simulink model "carpark_shuffler_sim"  (R2025b)
settings: Solver=VariableStepAuto  StartTime=0.0  StopTime=0.06  MaxStep=1e-4  RelTol=1e-4
PreLoadFcn:
  | init_params;
InitFcn:
  | init_params
undefined symbols (not defined in the file or in its folder): LOADP, SENSE, SRC
libraries: fl_lib x63, ee_lib x43, nesl_utility x37
(part 4 of 4)

== system carpark_shuffler_sim/Power Circuit/PV Module 1/power source/PV80 ==
  Diode : ee_lib/Semiconductors & Converters/Diode  ModelType=ee.enum.diode.modelType.pwl  TableType=ee.enum.diode.tableType.IfMat  IfMat=[.07, .12, .19, 1.75, 4.24, 7.32, 11.2; .16, .3, .72, 2.14, 5.02, 8.35, 13.12] A  VfMat=[.9, 1.15, 1.25, 1.5, 1.75, 2.17, 2.6, 2.85; .58, .68, .75, 1.1, 1.38, 1.77, 2.27, 2.7] V  TjVec=[25, 125] degC  VfVec=[.5, .7, .9, 1.3, 1.7, 2.1, 2.5] V  IfVec=[.1, .2, .5, 1, 2, 4, 7, 10] A  IrMat=[1e-06, 2e-06, 5e-06, 1e-05, 2.5e-05, 5e-05, .0001; 2e-06, 5e-06, 1e-05, 4e-05, 8e-05, .0002, .0005] A  VrMat=[10, 100, 200, 250, 300, 325, 350; 10, 70, 160, 220, 270, 300, 320] V  VrVec=[10, 20, 40, 50, 70, 80, 100] V  IrVec=[1e-06, 2e-06, 5e-06, 1e-05, 2e-05, 5e-05, .0001] A  Vf=0.6 V  Ron=0.3 Ohm  Goff=1e-8 S  prmExp=ee.enum.diode.expParam.useTwo  I12=[.0137, .545] A  V12=[.6, .7] V  RS=0 Ohm  Tmeas=298.15 K  IS=1e-12 A  ec=1  I1=0.0137 A  V1=0.6 V  N_series=1  N_parallel=1  ZenerEnable=false  Rz=0.3 Ohm  BV=inf V  C_param=ee.enum.diode.capParam.fixed  CJ=0 pF  CJ0=5 pF  Vvec=[.1, 10, 100] V  Cvec=[3.5, 1, .4] pF  VJ=1 V  Mgrad=0.5  FC=0.5  Q_param=ee.enum.diode.recoveryParam.off  iRM=-7.15 A  iF=4 A  didt=-750 A/us  trr_factor=3  trr=115 ns  Qrr=150 nA*s  Vr=-600 V  Ls=150 nH  Erec=0.03 J  TT=50 ns  tau=100 ns  T_param=ee.enum.diode.temperatureParam.off  Tdevice=298.15 K  I1_T2=0.245 A  V1_T2=0.5 V  IS_T2=1.25e-7 A  Tmeas2=125 degC  XTI_param=ee.enum.diode.xtiParam.pn  XTI=3  EG_param=ee.enum.diode.egapParam.material_si  EG=1.11 eV  dBVdT=0 V/K  enable_fault_input=simscape.enum.onoff.off  i_specify=off  i_priority=None  i=0 A  i_nominal_specify=off  i_nominal_value=1  i_nominal_unit=A  v_specify=off  v_priority=None  v=0 V  v_nominal_specify=off  v_nominal_value=1  v_nominal_unit=V  v_capacitor_specify=off  v_capacitor_priority=None  v_capacitor=0 V  v_capacitor_nominal_specify=off  v_capacitor_nominal_value=1  v_capacitor_nominal_unit=V  Qj_specify=off  Qj_priority=High  Qj=0 C  Qj_nominal_specify=off  Qj_nominal_value=1  Qj_nominal_unit=C  i_diode_specify=off  i_diode_priority=None  i_diode=0 A  i_diode_nominal_specify=off  i_diode_nominal_value=1  i_diode_nominal_unit=A  v_diode_specify=off  v_diode_priority=None  v_diode=0 V  v_diode_nominal_specify=off  v_diode_nominal_value=1  v_diode_nominal_unit=V  i_capacitor_specify=off  i_capacitor_priority=None  i_capacitor=0 A  i_capacitor_nominal_specify=off  i_capacitor_nominal_value=1  i_capacitor_nominal_unit=A  power_dissipated_specify=off  power_dissipated_priority=None  power_dissipated=0 W  power_dissipated_nominal_specify=off  power_dissipated_nominal_value=1  power_dissipated_nominal_unit=W  fidelity_level=ee.enum.diode.fidelity.includeChargeDyn  rec_loss_model=ee.enum.diode.reverseRecoveryModel.fixed  ErecVal=0 J  scaleWithIandV=true  ErecMat=zeros(2, 3) J  TjrecVec=[298.15, 398.15] K  IfrecVec=[.1, 1, 10] A  IrecVal=10 A  VrecVal=10 V  tFilter=1 / 1000 / 100 s  thermal_network_parameterization=ee.enum.thermalNetworkTopology.junctionCase  Rth=[0, 10] K/W  Rth_Cauer=[1, 3, 10] K/W  Rth_Foster=[.08, .14, .22, .16] K/W  thermal_mass_parameterization=ee.enum.thermalNetwork.timeconstant  thermal_mass=[0, 1] J/K  thermal_mass_Cauer=[.1, .3, 1] J/K  thermal_mass_Foster=[.001, .005, .05, .5] J/K  thermal_time_constant=[0, 10] s  thermal_time_constant_Cauer=[1, 3, 10] s  thermal_time_constant_Foster=[7e-05, .0007, .01, .08] s  thermal_mass_initial_temperatures=[25, 25] degC  thermal_mass_initial_temperatures_Cauer=[25, 25, 25] degC  junction_thermal_mass=0.01 J/K  Tvec_initial_Foster=[25, 25, 25, 25] degC  no_thermal_network=0  junction_temperature_specify=off  junction_temperature_priority=None  junction_temperature=25 degC  junction_temperature_nominal_specify=off  junction_temperature_nominal_value=1  junction_temperature_nominal_unit=degC
  Solar Cell : ee_lib/Sources/Solar Cell  prm=ee.enum.sources.solar_cell_prm.datasheet  Isc=SRC.pv80.Isc A  Voc=SRC.pv80.Voc_cell V  Is=1.728e-12 A  Is2=0 A  Iph=14.96 A  Ir0=1000 W/m^2  ec=1  N2=2  Rs=0.00263 Ohm  Rp=inf Ohm  N_series=SRC.pv80.Ns  N_parallel=1  TIPH1=0.0005 1/K  EG=1.11 eV  TXIS1=3  TXIS2=3  TRS1=0  TRP1=0  Tmeas=25 degC  TFIXED=25 degC  thermal_mass=100 J/K  initial_temperature=25 degC
  +ve : PMIOPort  Side=Left
  Irrad : PMIOPort  Port=2  Side=Left
  -ve : PMIOPort  Port=3  Side=Right
  connections:
  Solar Cell/LConn2 -- Diode/RConn1 -- +ve/RConn1
  -ve/RConn1 -- Solar Cell/RConn1 -- Diode/LConn1
  Irrad/RConn1 -- Solar Cell/LConn1

== system carpark_shuffler_sim/Power Circuit/PV Module 2/power source/BENCH ==
  Controlled Current Source : fl_lib/Electrical/Electrical Sources/Controlled Current Source
  DC Voltage Source : ee_lib/Additional Components/SPICE Sources/DC Voltage Source  DC=SRC.bench.Vset(1) V
  Diode : ee_lib/Semiconductors & Converters/Diode  ModelType=ee.enum.diode.modelType.pwl  TableType=ee.enum.diode.tableType.IfMat  IfMat=[.07, .12, .19, 1.75, 4.24, 7.32, 11.2; .16, .3, .72, 2.14, 5.02, 8.35, 13.12] A  VfMat=[.9, 1.15, 1.25, 1.5, 1.75, 2.17, 2.6, 2.85; .58, .68, .75, 1.1, 1.38, 1.77, 2.27, 2.7] V  TjVec=[25, 125] degC  VfVec=[.5, .7, .9, 1.3, 1.7, 2.1, 2.5] V  IfVec=[.1, .2, .5, 1, 2, 4, 7, 10] A  IrMat=[1e-06, 2e-06, 5e-06, 1e-05, 2.5e-05, 5e-05, .0001; 2e-06, 5e-06, 1e-05, 4e-05, 8e-05, .0002, .0005] A  VrMat=[10, 100, 200, 250, 300, 325, 350; 10, 70, 160, 220, 270, 300, 320] V  VrVec=[10, 20, 40, 50, 70, 80, 100] V  IrVec=[1e-06, 2e-06, 5e-06, 1e-05, 2e-05, 5e-05, .0001] A  Vf=1e-3 V  Ron=SRC.bench.Rclamp Ohm  Goff=1e-8 S  prmExp=ee.enum.diode.expParam.useTwo  I12=[.0137, .545] A  V12=[.6, .7] V  RS=0 Ohm  Tmeas=298.15 K  IS=1e-12 A  ec=1  I1=0.0137 A  V1=0.6 V  N_series=1  N_parallel=1  ZenerEnable=false  Rz=0.3 Ohm  BV=inf V  C_param=ee.enum.diode.capParam.fixed  CJ=0 pF  CJ0=5 pF  Vvec=[.1, 10, 100] V  Cvec=[3.5, 1, .4] pF  VJ=1 V  Mgrad=0.5  FC=0.5  Q_param=ee.enum.diode.recoveryParam.off  iRM=-7.15 A  iF=4 A  didt=-750 A/us  trr_factor=3  trr=115 ns  Qrr=150 nA*s  Vr=-600 V  Ls=150 nH  Erec=0.03 J  TT=50 ns  tau=100 ns  T_param=ee.enum.diode.temperatureParam.off  Tdevice=298.15 K  I1_T2=0.245 A  V1_T2=0.5 V  IS_T2=1.25e-7 A  Tmeas2=125 degC  XTI_param=ee.enum.diode.xtiParam.pn  XTI=3  EG_param=ee.enum.diode.egapParam.material_si  EG=1.11 eV  dBVdT=0 V/K  enable_fault_input=simscape.enum.onoff.off  i_specify=off  i_priority=None  i=0 A  i_nominal_specify=off  i_nominal_value=1  i_nominal_unit=A  v_specify=off  v_priority=None  v=0 V  v_nominal_specify=off  v_nominal_value=1  v_nominal_unit=V  v_capacitor_specify=off  v_capacitor_priority=None  v_capacitor=0 V  v_capacitor_nominal_specify=off  v_capacitor_nominal_value=1  v_capacitor_nominal_unit=V  Qj_specify=off  Qj_priority=High  Qj=0 C  Qj_nominal_specify=off  Qj_nominal_value=1  Qj_nominal_unit=C  i_diode_specify=off  i_diode_priority=None  i_diode=0 A  i_diode_nominal_specify=off  i_diode_nominal_value=1  i_diode_nominal_unit=A  v_diode_specify=off  v_diode_priority=None  v_diode=0 V  v_diode_nominal_specify=off  v_diode_nominal_value=1  v_diode_nominal_unit=V  i_capacitor_specify=off  i_capacitor_priority=None  i_capacitor=0 A  i_capacitor_nominal_specify=off  i_capacitor_nominal_value=1  i_capacitor_nominal_unit=A  power_dissipated_specify=off  power_dissipated_priority=None  power_dissipated=0 W  power_dissipated_nominal_specify=off  power_dissipated_nominal_value=1  power_dissipated_nominal_unit=W  fidelity_level=ee.enum.diode.fidelity.includeChargeDyn  rec_loss_model=ee.enum.diode.reverseRecoveryModel.fixed  ErecVal=0 J  scaleWithIandV=true  ErecMat=zeros(2, 3) J  TjrecVec=[298.15, 398.15] K  IfrecVec=[.1, 1, 10] A  IrecVal=10 A  VrecVal=10 V  tFilter=1 / 1000 / 100 s  thermal_network_parameterization=ee.enum.thermalNetworkTopology.junctionCase  Rth=[0, 10] K/W  Rth_Cauer=[1, 3, 10] K/W  Rth_Foster=[.08, .14, .22, .16] K/W  thermal_mass_parameterization=ee.enum.thermalNetwork.timeconstant  thermal_mass=[0, 1] J/K  thermal_mass_Cauer=[.1, .3, 1] J/K  thermal_mass_Foster=[.001, .005, .05, .5] J/K  thermal_time_constant=[0, 10] s  thermal_time_constant_Cauer=[1, 3, 10] s  thermal_time_constant_Foster=[7e-05, .0007, .01, .08] s  thermal_mass_initial_temperatures=[25, 25] degC  thermal_mass_initial_temperatures_Cauer=[25, 25, 25] degC  junction_thermal_mass=0.01 J/K  Tvec_initial_Foster=[25, 25, 25, 25] degC  no_thermal_network=0  junction_temperature_specify=off  junction_temperature_priority=None  junction_temperature=25 degC  junction_temperature_nominal_specify=off  junction_temperature_nominal_value=1  junction_temperature_nominal_unit=degC
  PS Gain : fl_lib/Physical Signals/Functions/PS Gain  gain=SRC.bench.Ilim(2)/1000
  Resistor : fl_lib/Electrical/Electrical Elements/Resistor  R=max(SRC.bench.Rs(1),1e-6) Ohm  i_specify=off  i_priority=None  i=0 A  i_nominal_specify=off  i_nominal_value=1  i_nominal_unit=A  v_specify=off  v_priority=None  v=0 V  v_nominal_specify=off  v_nominal_value=1  v_nominal_unit=V
  +ve : PMIOPort  Side=Left
  Irrad : PMIOPort  Port=2  Side=Left
  -ve : PMIOPort  Port=3  Side=Right
  connections:
  Resistor/RConn1 -- +ve/RConn1
  Controlled Current Source/RConn2 -- -ve/RConn1 -- DC Voltage Source/RConn1
  PS Gain/RConn1 -- Controlled Current Source/RConn1
  Controlled Current Source/LConn1 -- Resistor/LConn1 -- Diode/LConn1
  DC Voltage Source/LConn1 -- Diode/RConn1
  PS Gain/LConn1 -- Irrad/RConn1

== system carpark_shuffler_sim/Power Circuit/PV Module 2/power source/PV80 ==
  Diode : ee_lib/Semiconductors & Converters/Diode  ModelType=ee.enum.diode.modelType.pwl  TableType=ee.enum.diode.tableType.IfMat  IfMat=[.07, .12, .19, 1.75, 4.24, 7.32, 11.2; .16, .3, .72, 2.14, 5.02, 8.35, 13.12] A  VfMat=[.9, 1.15, 1.25, 1.5, 1.75, 2.17, 2.6, 2.85; .58, .68, .75, 1.1, 1.38, 1.77, 2.27, 2.7] V  TjVec=[25, 125] degC  VfVec=[.5, .7, .9, 1.3, 1.7, 2.1, 2.5] V  IfVec=[.1, .2, .5, 1, 2, 4, 7, 10] A  IrMat=[1e-06, 2e-06, 5e-06, 1e-05, 2.5e-05, 5e-05, .0001; 2e-06, 5e-06, 1e-05, 4e-05, 8e-05, .0002, .0005] A  VrMat=[10, 100, 200, 250, 300, 325, 350; 10, 70, 160, 220, 270, 300, 320] V  VrVec=[10, 20, 40, 50, 70, 80, 100] V  IrVec=[1e-06, 2e-06, 5e-06, 1e-05, 2e-05, 5e-05, .0001] A  Vf=0.6 V  Ron=0.3 Ohm  Goff=1e-8 S  prmExp=ee.enum.diode.expParam.useTwo  I12=[.0137, .545] A  V12=[.6, .7] V  RS=0 Ohm  Tmeas=298.15 K  IS=1e-12 A  ec=1  I1=0.0137 A  V1=0.6 V  N_series=1  N_parallel=1  ZenerEnable=false  Rz=0.3 Ohm  BV=inf V  C_param=ee.enum.diode.capParam.fixed  CJ=0 pF  CJ0=5 pF  Vvec=[.1, 10, 100] V  Cvec=[3.5, 1, .4] pF  VJ=1 V  Mgrad=0.5  FC=0.5  Q_param=ee.enum.diode.recoveryParam.off  iRM=-7.15 A  iF=4 A  didt=-750 A/us  trr_factor=3  trr=115 ns  Qrr=150 nA*s  Vr=-600 V  Ls=150 nH  Erec=0.03 J  TT=50 ns  tau=100 ns  T_param=ee.enum.diode.temperatureParam.off  Tdevice=298.15 K  I1_T2=0.245 A  V1_T2=0.5 V  IS_T2=1.25e-7 A  Tmeas2=125 degC  XTI_param=ee.enum.diode.xtiParam.pn  XTI=3  EG_param=ee.enum.diode.egapParam.material_si  EG=1.11 eV  dBVdT=0 V/K  enable_fault_input=simscape.enum.onoff.off  i_specify=off  i_priority=None  i=0 A  i_nominal_specify=off  i_nominal_value=1  i_nominal_unit=A  v_specify=off  v_priority=None  v=0 V  v_nominal_specify=off  v_nominal_value=1  v_nominal_unit=V  v_capacitor_specify=off  v_capacitor_priority=None  v_capacitor=0 V  v_capacitor_nominal_specify=off  v_capacitor_nominal_value=1  v_capacitor_nominal_unit=V  Qj_specify=off  Qj_priority=High  Qj=0 C  Qj_nominal_specify=off  Qj_nominal_value=1  Qj_nominal_unit=C  i_diode_specify=off  i_diode_priority=None  i_diode=0 A  i_diode_nominal_specify=off  i_diode_nominal_value=1  i_diode_nominal_unit=A  v_diode_specify=off  v_diode_priority=None  v_diode=0 V  v_diode_nominal_specify=off  v_diode_nominal_value=1  v_diode_nominal_unit=V  i_capacitor_specify=off  i_capacitor_priority=None  i_capacitor=0 A  i_capacitor_nominal_specify=off  i_capacitor_nominal_value=1  i_capacitor_nominal_unit=A  power_dissipated_specify=off  power_dissipated_priority=None  power_dissipated=0 W  power_dissipated_nominal_specify=off  power_dissipated_nominal_value=1  power_dissipated_nominal_unit=W  fidelity_level=ee.enum.diode.fidelity.includeChargeDyn  rec_loss_model=ee.enum.diode.reverseRecoveryModel.fixed  ErecVal=0 J  scaleWithIandV=true  ErecMat=zeros(2, 3) J  TjrecVec=[298.15, 398.15] K  IfrecVec=[.1, 1, 10] A  IrecVal=10 A  VrecVal=10 V  tFilter=1 / 1000 / 100 s  thermal_network_parameterization=ee.enum.thermalNetworkTopology.junctionCase  Rth=[0, 10] K/W  Rth_Cauer=[1, 3, 10] K/W  Rth_Foster=[.08, .14, .22, .16] K/W  thermal_mass_parameterization=ee.enum.thermalNetwork.timeconstant  thermal_mass=[0, 1] J/K  thermal_mass_Cauer=[.1, .3, 1] J/K  thermal_mass_Foster=[.001, .005, .05, .5] J/K  thermal_time_constant=[0, 10] s  thermal_time_constant_Cauer=[1, 3, 10] s  thermal_time_constant_Foster=[7e-05, .0007, .01, .08] s  thermal_mass_initial_temperatures=[25, 25] degC  thermal_mass_initial_temperatures_Cauer=[25, 25, 25] degC  junction_thermal_mass=0.01 J/K  Tvec_initial_Foster=[25, 25, 25, 25] degC  no_thermal_network=0  junction_temperature_specify=off  junction_temperature_priority=None  junction_temperature=25 degC  junction_temperature_nominal_specify=off  junction_temperature_nominal_value=1  junction_temperature_nominal_unit=degC
  Solar Cell : ee_lib/Sources/Solar Cell  prm=ee.enum.sources.solar_cell_prm.datasheet  Isc=SRC.pv80.Isc A  Voc=SRC.pv80.Voc_cell V  Is=1.728e-12 A  Is2=0 A  Iph=14.96 A  Ir0=1000 W/m^2  ec=1  N2=2  Rs=0.00263 Ohm  Rp=inf Ohm  N_series=SRC.pv80.Ns  N_parallel=1  TIPH1=0.0005 1/K  EG=1.11 eV  TXIS1=3  TXIS2=3  TRS1=0  TRP1=0  Tmeas=25 degC  TFIXED=25 degC  thermal_mass=100 J/K  initial_temperature=25 degC
  +ve : PMIOPort  Side=Left
  Irrad : PMIOPort  Port=2  Side=Left
  -ve : PMIOPort  Port=3  Side=Right
  connections:
  Diode/RConn1 -- Solar Cell/LConn2 -- +ve/RConn1
  Diode/LConn1 -- -ve/RConn1 -- Solar Cell/RConn1
  Irrad/RConn1 -- Solar Cell/LConn1

== system carpark_shuffler_sim/Power Circuit/PV Module 3/power source/BENCH ==
  Controlled Current Source : fl_lib/Electrical/Electrical Sources/Controlled Current Source
  DC Voltage Source : ee_lib/Additional Components/SPICE Sources/DC Voltage Source  DC=SRC.bench.Vset(1) V
  Diode : ee_lib/Semiconductors & Converters/Diode  ModelType=ee.enum.diode.modelType.pwl  TableType=ee.enum.diode.tableType.IfMat  IfMat=[.07, .12, .19, 1.75, 4.24, 7.32, 11.2; .16, .3, .72, 2.14, 5.02, 8.35, 13.12] A  VfMat=[.9, 1.15, 1.25, 1.5, 1.75, 2.17, 2.6, 2.85; .58, .68, .75, 1.1, 1.38, 1.77, 2.27, 2.7] V  TjVec=[25, 125] degC  VfVec=[.5, .7, .9, 1.3, 1.7, 2.1, 2.5] V  IfVec=[.1, .2, .5, 1, 2, 4, 7, 10] A  IrMat=[1e-06, 2e-06, 5e-06, 1e-05, 2.5e-05, 5e-05, .0001; 2e-06, 5e-06, 1e-05, 4e-05, 8e-05, .0002, .0005] A  VrMat=[10, 100, 200, 250, 300, 325, 350; 10, 70, 160, 220, 270, 300, 320] V  VrVec=[10, 20, 40, 50, 70, 80, 100] V  IrVec=[1e-06, 2e-06, 5e-06, 1e-05, 2e-05, 5e-05, .0001] A  Vf=1e-3 V  Ron=SRC.bench.Rclamp Ohm  Goff=1e-8 S  prmExp=ee.enum.diode.expParam.useTwo  I12=[.0137, .545] A  V12=[.6, .7] V  RS=0 Ohm  Tmeas=298.15 K  IS=1e-12 A  ec=1  I1=0.0137 A  V1=0.6 V  N_series=1  N_parallel=1  ZenerEnable=false  Rz=0.3 Ohm  BV=inf V  C_param=ee.enum.diode.capParam.fixed  CJ=0 pF  CJ0=5 pF  Vvec=[.1, 10, 100] V  Cvec=[3.5, 1, .4] pF  VJ=1 V  Mgrad=0.5  FC=0.5  Q_param=ee.enum.diode.recoveryParam.off  iRM=-7.15 A  iF=4 A  didt=-750 A/us  trr_factor=3  trr=115 ns  Qrr=150 nA*s  Vr=-600 V  Ls=150 nH  Erec=0.03 J  TT=50 ns  tau=100 ns  T_param=ee.enum.diode.temperatureParam.off  Tdevice=298.15 K  I1_T2=0.245 A  V1_T2=0.5 V  IS_T2=1.25e-7 A  Tmeas2=125 degC  XTI_param=ee.enum.diode.xtiParam.pn  XTI=3  EG_param=ee.enum.diode.egapParam.material_si  EG=1.11 eV  dBVdT=0 V/K  enable_fault_input=simscape.enum.onoff.off  i_specify=off  i_priority=None  i=0 A  i_nominal_specify=off  i_nominal_value=1  i_nominal_unit=A  v_specify=off  v_priority=None  v=0 V  v_nominal_specify=off  v_nominal_value=1  v_nominal_unit=V  v_capacitor_specify=off  v_capacitor_priority=None  v_capacitor=0 V  v_capacitor_nominal_specify=off  v_capacitor_nominal_value=1  v_capacitor_nominal_unit=V  Qj_specify=off  Qj_priority=High  Qj=0 C  Qj_nominal_specify=off  Qj_nominal_value=1  Qj_nominal_unit=C  i_diode_specify=off  i_diode_priority=None  i_diode=0 A  i_diode_nominal_specify=off  i_diode_nominal_value=1  i_diode_nominal_unit=A  v_diode_specify=off  v_diode_priority=None  v_diode=0 V  v_diode_nominal_specify=off  v_diode_nominal_value=1  v_diode_nominal_unit=V  i_capacitor_specify=off  i_capacitor_priority=None  i_capacitor=0 A  i_capacitor_nominal_specify=off  i_capacitor_nominal_value=1  i_capacitor_nominal_unit=A  power_dissipated_specify=off  power_dissipated_priority=None  power_dissipated=0 W  power_dissipated_nominal_specify=off  power_dissipated_nominal_value=1  power_dissipated_nominal_unit=W  fidelity_level=ee.enum.diode.fidelity.includeChargeDyn  rec_loss_model=ee.enum.diode.reverseRecoveryModel.fixed  ErecVal=0 J  scaleWithIandV=true  ErecMat=zeros(2, 3) J  TjrecVec=[298.15, 398.15] K  IfrecVec=[.1, 1, 10] A  IrecVal=10 A  VrecVal=10 V  tFilter=1 / 1000 / 100 s  thermal_network_parameterization=ee.enum.thermalNetworkTopology.junctionCase  Rth=[0, 10] K/W  Rth_Cauer=[1, 3, 10] K/W  Rth_Foster=[.08, .14, .22, .16] K/W  thermal_mass_parameterization=ee.enum.thermalNetwork.timeconstant  thermal_mass=[0, 1] J/K  thermal_mass_Cauer=[.1, .3, 1] J/K  thermal_mass_Foster=[.001, .005, .05, .5] J/K  thermal_time_constant=[0, 10] s  thermal_time_constant_Cauer=[1, 3, 10] s  thermal_time_constant_Foster=[7e-05, .0007, .01, .08] s  thermal_mass_initial_temperatures=[25, 25] degC  thermal_mass_initial_temperatures_Cauer=[25, 25, 25] degC  junction_thermal_mass=0.01 J/K  Tvec_initial_Foster=[25, 25, 25, 25] degC  no_thermal_network=0  junction_temperature_specify=off  junction_temperature_priority=None  junction_temperature=25 degC  junction_temperature_nominal_specify=off  junction_temperature_nominal_value=1  junction_temperature_nominal_unit=degC
  PS Gain : fl_lib/Physical Signals/Functions/PS Gain  gain=SRC.bench.Ilim(3)/1000
  Resistor : fl_lib/Electrical/Electrical Elements/Resistor  R=max(SRC.bench.Rs(1),1e-6) Ohm  i_specify=off  i_priority=None  i=0 A  i_nominal_specify=off  i_nominal_value=1  i_nominal_unit=A  v_specify=off  v_priority=None  v=0 V  v_nominal_specify=off  v_nominal_value=1  v_nominal_unit=V
  +ve : PMIOPort  Side=Left
  Irrad : PMIOPort  Port=2  Side=Left
  -ve : PMIOPort  Port=3  Side=Right
  connections:
  Resistor/RConn1 -- +ve/RConn1
  Controlled Current Source/RConn2 -- -ve/RConn1 -- DC Voltage Source/RConn1
  PS Gain/RConn1 -- Controlled Current Source/RConn1
  Controlled Current Source/LConn1 -- Resistor/LConn1 -- Diode/LConn1
  DC Voltage Source/LConn1 -- Diode/RConn1
  PS Gain/LConn1 -- Irrad/RConn1

== system carpark_shuffler_sim/Power Circuit/PV Module 3/power source/PV80 ==
  Diode : ee_lib/Semiconductors & Converters/Diode  ModelType=ee.enum.diode.modelType.pwl  TableType=ee.enum.diode.tableType.IfMat  IfMat=[.07, .12, .19, 1.75, 4.24, 7.32, 11.2; .16, .3, .72, 2.14, 5.02, 8.35, 13.12] A  VfMat=[.9, 1.15, 1.25, 1.5, 1.75, 2.17, 2.6, 2.85; .58, .68, .75, 1.1, 1.38, 1.77, 2.27, 2.7] V  TjVec=[25, 125] degC  VfVec=[.5, .7, .9, 1.3, 1.7, 2.1, 2.5] V  IfVec=[.1, .2, .5, 1, 2, 4, 7, 10] A  IrMat=[1e-06, 2e-06, 5e-06, 1e-05, 2.5e-05, 5e-05, .0001; 2e-06, 5e-06, 1e-05, 4e-05, 8e-05, .0002, .0005] A  VrMat=[10, 100, 200, 250, 300, 325, 350; 10, 70, 160, 220, 270, 300, 320] V  VrVec=[10, 20, 40, 50, 70, 80, 100] V  IrVec=[1e-06, 2e-06, 5e-06, 1e-05, 2e-05, 5e-05, .0001] A  Vf=0.6 V  Ron=0.3 Ohm  Goff=1e-8 S  prmExp=ee.enum.diode.expParam.useTwo  I12=[.0137, .545] A  V12=[.6, .7] V  RS=0 Ohm  Tmeas=298.15 K  IS=1e-12 A  ec=1  I1=0.0137 A  V1=0.6 V  N_series=1  N_parallel=1  ZenerEnable=false  Rz=0.3 Ohm  BV=inf V  C_param=ee.enum.diode.capParam.fixed  CJ=0 pF  CJ0=5 pF  Vvec=[.1, 10, 100] V  Cvec=[3.5, 1, .4] pF  VJ=1 V  Mgrad=0.5  FC=0.5  Q_param=ee.enum.diode.recoveryParam.off  iRM=-7.15 A  iF=4 A  didt=-750 A/us  trr_factor=3  trr=115 ns  Qrr=150 nA*s  Vr=-600 V  Ls=150 nH  Erec=0.03 J  TT=50 ns  tau=100 ns  T_param=ee.enum.diode.temperatureParam.off  Tdevice=298.15 K  I1_T2=0.245 A  V1_T2=0.5 V  IS_T2=1.25e-7 A  Tmeas2=125 degC  XTI_param=ee.enum.diode.xtiParam.pn  XTI=3  EG_param=ee.enum.diode.egapParam.material_si  EG=1.11 eV  dBVdT=0 V/K  enable_fault_input=simscape.enum.onoff.off  i_specify=off  i_priority=None  i=0 A  i_nominal_specify=off  i_nominal_value=1  i_nominal_unit=A  v_specify=off  v_priority=None  v=0 V  v_nominal_specify=off  v_nominal_value=1  v_nominal_unit=V  v_capacitor_specify=off  v_capacitor_priority=None  v_capacitor=0 V  v_capacitor_nominal_specify=off  v_capacitor_nominal_value=1  v_capacitor_nominal_unit=V  Qj_specify=off  Qj_priority=High  Qj=0 C  Qj_nominal_specify=off  Qj_nominal_value=1  Qj_nominal_unit=C  i_diode_specify=off  i_diode_priority=None  i_diode=0 A  i_diode_nominal_specify=off  i_diode_nominal_value=1  i_diode_nominal_unit=A  v_diode_specify=off  v_diode_priority=None  v_diode=0 V  v_diode_nominal_specify=off  v_diode_nominal_value=1  v_diode_nominal_unit=V  i_capacitor_specify=off  i_capacitor_priority=None  i_capacitor=0 A  i_capacitor_nominal_specify=off  i_capacitor_nominal_value=1  i_capacitor_nominal_unit=A  power_dissipated_specify=off  power_dissipated_priority=None  power_dissipated=0 W  power_dissipated_nominal_specify=off  power_dissipated_nominal_value=1  power_dissipated_nominal_unit=W  fidelity_level=ee.enum.diode.fidelity.includeChargeDyn  rec_loss_model=ee.enum.diode.reverseRecoveryModel.fixed  ErecVal=0 J  scaleWithIandV=true  ErecMat=zeros(2, 3) J  TjrecVec=[298.15, 398.15] K  IfrecVec=[.1, 1, 10] A  IrecVal=10 A  VrecVal=10 V  tFilter=1 / 1000 / 100 s  thermal_network_parameterization=ee.enum.thermalNetworkTopology.junctionCase  Rth=[0, 10] K/W  Rth_Cauer=[1, 3, 10] K/W  Rth_Foster=[.08, .14, .22, .16] K/W  thermal_mass_parameterization=ee.enum.thermalNetwork.timeconstant  thermal_mass=[0, 1] J/K  thermal_mass_Cauer=[.1, .3, 1] J/K  thermal_mass_Foster=[.001, .005, .05, .5] J/K  thermal_time_constant=[0, 10] s  thermal_time_constant_Cauer=[1, 3, 10] s  thermal_time_constant_Foster=[7e-05, .0007, .01, .08] s  thermal_mass_initial_temperatures=[25, 25] degC  thermal_mass_initial_temperatures_Cauer=[25, 25, 25] degC  junction_thermal_mass=0.01 J/K  Tvec_initial_Foster=[25, 25, 25, 25] degC  no_thermal_network=0  junction_temperature_specify=off  junction_temperature_priority=None  junction_temperature=25 degC  junction_temperature_nominal_specify=off  junction_temperature_nominal_value=1  junction_temperature_nominal_unit=degC
  Solar Cell : ee_lib/Sources/Solar Cell  prm=ee.enum.sources.solar_cell_prm.datasheet  Isc=SRC.pv80.Isc A  Voc=SRC.pv80.Voc_cell V  Is=1.728e-12 A  Is2=0 A  Iph=14.96 A  Ir0=1000 W/m^2  ec=1  N2=2  Rs=0.00263 Ohm  Rp=inf Ohm  N_series=SRC.pv80.Ns  N_parallel=1  TIPH1=0.0005 1/K  EG=1.11 eV  TXIS1=3  TXIS2=3  TRS1=0  TRP1=0  Tmeas=25 degC  TFIXED=25 degC  thermal_mass=100 J/K  initial_temperature=25 degC
  +ve : PMIOPort  Side=Left
  Irrad : PMIOPort  Port=2  Side=Left
  -ve : PMIOPort  Port=3  Side=Right
  connections:
  Diode/RConn1 -- Solar Cell/LConn2 -- +ve/RConn1
  Diode/LConn1 -- -ve/RConn1 -- Solar Cell/RConn1
  Irrad/RConn1 -- Solar Cell/LConn1

== system carpark_shuffler_sim/Power Circuit/Power Shuffler1/Phase A Half Bridge/Phase A Gate Driver ==
  A Control : Inport
  Controlled PWM Voltage : ee_lib/Integrated Circuits/Controlled PWM Voltage  F=200 kHz  TD=0 s  pulse_width_offset=0 s  pulse_min=0 s  pwm_or_av=ee.enum.pwm_or_av.pwm  event_type=ee.enum.ic.event.asynchronous  sample_time=1e-6 s  Vmin=0 V  Vmax=5 V  Vm=5 V  u_min=0  u_max=1
      settings: InternalSimscapePortConfiguration="{\"Bottom\":[],\"Left\":[{\"id\":\"u\",\"label\":\"u\",\"type\":\"input\"}],\"Right\":[{\"id\":\"p2\",\"label\":\"PWM\",\"type\":\"foundation.electrical.electrical\"},{\"id\":\"n2\",\"label\":\"REF\",\"type\":\"foundation.electrical.electrical\"}],\"Top\":[]}"
  Electrical Reference : fl_lib/Electrical/Electrical Elements/Electrical Reference
  Electrical Reference1 : fl_lib/Electrical/Electrical Elements/Electrical Reference
  Half-Bridge Driver : ee_lib/Semiconductors & Converters/Half-Bridge Driver  port_option=ee.enum.controlport.elec  uHigh=2.0 V  uLow=0.8 V  uHighValue=0.7  uLowValue=0.3  vHigh=15 V  vLow=0 V  tpLH=50 ns  tdLH=100 ns  tpHL=50 ns  tdHL=100 ns  parameterization=ee.enum.semiconductors.gateDriverParam.outputImpedance  rHigh=2 Ohm  rLow=2 Ohm  tRise=20 ns  tFall=20 ns  cLoad=10 nF  ZonTime_specify=off  ZonTime_priority=None  ZonTime=0 s  ZoffTime_specify=off  ZoffTime_priority=None  ZoffTime=0 s  power_dissipated_high_side_specify=off  power_dissipated_high_side_priority=None  power_dissipated_high_side=0 W  power_dissipated_high_side_nominal_specify=off  power_dissipated_high_side_nominal_value=1  power_dissipated_high_side_nominal_unit=W  power_dissipated_low_side_specify=off  power_dissipated_low_side_priority=None  power_dissipated_low_side=0 W  power_dissipated_low_side_nominal_specify=off  power_dissipated_low_side_nominal_value=1  power_dissipated_low_side_nominal_unit=W
      settings: InternalSimscapePortConfiguration="{\"Bottom\":[],\"Left\":[{\"id\":\"PWM\",\"label\":\"PWM\",\"type\":\"foundation.electrical.electrical\"},{\"id\":\"REF\",\"label\":\"REF\",\"type\":\"foundation.electrical.electrical\"}],\"Right\":[{\"id\":\"HO\",\"label\":\"HO\",\"type\":\"foundation.electrical.electrical\"},{\"id\":\"HS\",\"label\":\"HS\",\"type\":\"foundation.electrical.electrical\"},{\"id\":\"LO\",\"label\":\"LO\",\"type\":\"foundation.electrical.electrical\"},{\"id\":\"LS\",\"label\":\"LS\",\"type\":\"foundation.electrical.electrical\"}],\"Top\":[]}"
  Simulink-PS Converter1 : nesl_utility/Simulink-PS Converter  PhysicalDomain=network_engine_domain  SubClassName=ps_input  LeftPortType=input  RightPortType=output  PseudoPeriodic=off  Frequencies=[]  NoiseDistribution=none  NoiseParameters=[]  Unit=1  AffineConversion=off  FilteringAndDerivatives=provide  SimscapeFilterOrder=1  InputFilterTimeConstant=0.001  UdotUserProvided=0
  PWMH : PMIOPort  Side=Right
  phase : PMIOPort  Port=2  Side=Right
  PWML : PMIOPort  Port=3  Side=Right
  wires:
  A Control/1 -> Simulink-PS Converter1/1
  connections:
  Half-Bridge Driver/LConn2 -- Electrical Reference1/LConn1 -- Controlled PWM Voltage/RConn2
  Simulink-PS Converter1/RConn1 -- Controlled PWM Voltage/LConn1
  Half-Bridge Driver/RConn3 -- PWML/RConn1
  Electrical Reference/LConn1 -- Half-Bridge Driver/RConn4
  Half-Bridge Driver/RConn2 -- phase/RConn1
  Half-Bridge Driver/RConn1 -- PWMH/RConn1
  Controlled PWM Voltage/RConn1 -- Half-Bridge Driver/LConn1

== system carpark_shuffler_sim/Power Circuit/Power Shuffler1/Phase B Half Bridge/Phase B Gate Driver ==
  B Control : Inport
  Controlled PWM Voltage : ee_lib/Integrated Circuits/Controlled PWM Voltage  F=200 kHz  TD=1/(2 *200000) s  pulse_width_offset=0 s  pulse_min=0 s  pwm_or_av=ee.enum.pwm_or_av.pwm  event_type=ee.enum.ic.event.asynchronous  sample_time=1e-6 s  Vmin=0 V  Vmax=5 V  Vm=5 V  u_min=0  u_max=1
      settings: InternalSimscapePortConfiguration="{\"Bottom\":[],\"Left\":[{\"id\":\"u\",\"label\":\"u\",\"type\":\"input\"}],\"Right\":[{\"id\":\"p2\",\"label\":\"PWM\",\"type\":\"foundation.electrical.electrical\"},{\"id\":\"n2\",\"label\":\"REF\",\"type\":\"foundation.electrical.electrical\"}],\"Top\":[]}"
  Electrical Reference : fl_lib/Electrical/Electrical Elements/Electrical Reference
  Electrical Reference1 : fl_lib/Electrical/Electrical Elements/Electrical Reference
  Half-Bridge Driver : ee_lib/Semiconductors & Converters/Half-Bridge Driver  port_option=ee.enum.controlport.elec  uHigh=2.0 V  uLow=0.8 V  uHighValue=0.7  uLowValue=0.3  vHigh=15 V  vLow=0 V  tpLH=50 ns  tdLH=100 ns  tpHL=50 ns  tdHL=100 ns  parameterization=ee.enum.semiconductors.gateDriverParam.outputImpedance  rHigh=2 Ohm  rLow=2 Ohm  tRise=20 ns  tFall=20 ns  cLoad=10 nF  ZonTime_specify=off  ZonTime_priority=None  ZonTime=0 s  ZoffTime_specify=off  ZoffTime_priority=None  ZoffTime=0 s  power_dissipated_high_side_specify=off  power_dissipated_high_side_priority=None  power_dissipated_high_side=0 W  power_dissipated_high_side_nominal_specify=off  power_dissipated_high_side_nominal_value=1  power_dissipated_high_side_nominal_unit=W  power_dissipated_low_side_specify=off  power_dissipated_low_side_priority=None  power_dissipated_low_side=0 W  power_dissipated_low_side_nominal_specify=off  power_dissipated_low_side_nominal_value=1  power_dissipated_low_side_nominal_unit=W
      settings: InternalSimscapePortConfiguration="{\"Bottom\":[],\"Left\":[{\"id\":\"PWM\",\"label\":\"PWM\",\"type\":\"foundation.electrical.electrical\"},{\"id\":\"REF\",\"label\":\"REF\",\"type\":\"foundation.electrical.electrical\"}],\"Right\":[{\"id\":\"HO\",\"label\":\"HO\",\"type\":\"foundation.electrical.electrical\"},{\"id\":\"HS\",\"label\":\"HS\",\"type\":\"foundation.electrical.electrical\"},{\"id\":\"LO\",\"label\":\"LO\",\"type\":\"foundation.electrical.electrical\"},{\"id\":\"LS\",\"label\":\"LS\",\"type\":\"foundation.electrical.electrical\"}],\"Top\":[]}"
  Simulink-PS Converter1 : nesl_utility/Simulink-PS Converter  PhysicalDomain=network_engine_domain  SubClassName=ps_input  LeftPortType=input  RightPortType=output  PseudoPeriodic=off  Frequencies=[]  NoiseDistribution=none  NoiseParameters=[]  Unit=1  AffineConversion=off  FilteringAndDerivatives=provide  SimscapeFilterOrder=1  InputFilterTimeConstant=0.001  UdotUserProvided=0
  PWMH : PMIOPort  Side=Right
  phase : PMIOPort  Port=2  Side=Right
  PWML : PMIOPort  Port=3  Side=Right
  wires:
  B Control/1 -> Simulink-PS Converter1/1
  connections:
  Half-Bridge Driver/RConn2 -- phase/RConn1
  Half-Bridge Driver/RConn1 -- PWMH/RConn1
  Half-Bridge Driver/RConn3 -- PWML/RConn1
  Electrical Reference/LConn1 -- Half-Bridge Driver/RConn4
  Simulink-PS Converter1/RConn1 -- Controlled PWM Voltage/LConn1
  Controlled PWM Voltage/RConn1 -- Half-Bridge Driver/LConn1
  Electrical Reference1/LConn1 -- Controlled PWM Voltage/RConn2 -- Half-Bridge Driver/LConn2

== system carpark_shuffler_sim/Power Circuit/Power Shuffler2/Phase A Half Bridge/Phase A Gate Driver ==
  A Control : Inport
  Controlled PWM Voltage : ee_lib/Integrated Circuits/Controlled PWM Voltage  F=200 kHz  TD=0 s  pulse_width_offset=0 s  pulse_min=0 s  pwm_or_av=ee.enum.pwm_or_av.pwm  event_type=ee.enum.ic.event.asynchronous  sample_time=1e-6 s  Vmin=0 V  Vmax=5 V  Vm=5 V  u_min=0  u_max=1
      settings: InternalSimscapePortConfiguration="{\"Bottom\":[],\"Left\":[{\"id\":\"u\",\"label\":\"u\",\"type\":\"input\"}],\"Right\":[{\"id\":\"p2\",\"label\":\"PWM\",\"type\":\"foundation.electrical.electrical\"},{\"id\":\"n2\",\"label\":\"REF\",\"type\":\"foundation.electrical.electrical\"}],\"Top\":[]}"
  Electrical Reference : fl_lib/Electrical/Electrical Elements/Electrical Reference
  Electrical Reference1 : fl_lib/Electrical/Electrical Elements/Electrical Reference
  Half-Bridge Driver : ee_lib/Semiconductors & Converters/Half-Bridge Driver  port_option=ee.enum.controlport.elec  uHigh=2.0 V  uLow=0.8 V  uHighValue=0.7  uLowValue=0.3  vHigh=15 V  vLow=0 V  tpLH=50 ns  tdLH=100 ns  tpHL=50 ns  tdHL=100 ns  parameterization=ee.enum.semiconductors.gateDriverParam.outputImpedance  rHigh=2 Ohm  rLow=2 Ohm  tRise=20 ns  tFall=20 ns  cLoad=10 nF  ZonTime_specify=off  ZonTime_priority=None  ZonTime=0 s  ZoffTime_specify=off  ZoffTime_priority=None  ZoffTime=0 s  power_dissipated_high_side_specify=off  power_dissipated_high_side_priority=None  power_dissipated_high_side=0 W  power_dissipated_high_side_nominal_specify=off  power_dissipated_high_side_nominal_value=1  power_dissipated_high_side_nominal_unit=W  power_dissipated_low_side_specify=off  power_dissipated_low_side_priority=None  power_dissipated_low_side=0 W  power_dissipated_low_side_nominal_specify=off  power_dissipated_low_side_nominal_value=1  power_dissipated_low_side_nominal_unit=W
      settings: InternalSimscapePortConfiguration="{\"Bottom\":[],\"Left\":[{\"id\":\"PWM\",\"label\":\"PWM\",\"type\":\"foundation.electrical.electrical\"},{\"id\":\"REF\",\"label\":\"REF\",\"type\":\"foundation.electrical.electrical\"}],\"Right\":[{\"id\":\"HO\",\"label\":\"HO\",\"type\":\"foundation.electrical.electrical\"},{\"id\":\"HS\",\"label\":\"HS\",\"type\":\"foundation.electrical.electrical\"},{\"id\":\"LO\",\"label\":\"LO\",\"type\":\"foundation.electrical.electrical\"},{\"id\":\"LS\",\"label\":\"LS\",\"type\":\"foundation.electrical.electrical\"}],\"Top\":[]}"
  Simulink-PS Converter1 : nesl_utility/Simulink-PS Converter  PhysicalDomain=network_engine_domain  SubClassName=ps_input  LeftPortType=input  RightPortType=output  PseudoPeriodic=off  Frequencies=[]  NoiseDistribution=none  NoiseParameters=[]  Unit=1  AffineConversion=off  FilteringAndDerivatives=provide  SimscapeFilterOrder=1  InputFilterTimeConstant=0.001  UdotUserProvided=0
  PWMH : PMIOPort  Side=Right
  phase : PMIOPort  Port=2  Side=Right
  PWML : PMIOPort  Port=3  Side=Right
  wires:
  A Control/1 -> Simulink-PS Converter1/1
  connections:
  Half-Bridge Driver/LConn2 -- Electrical Reference1/LConn1 -- Controlled PWM Voltage/RConn2
  Simulink-PS Converter1/RConn1 -- Controlled PWM Voltage/LConn1
  Half-Bridge Driver/RConn3 -- PWML/RConn1
  Electrical Reference/LConn1 -- Half-Bridge Driver/RConn4
  Half-Bridge Driver/RConn2 -- phase/RConn1
  Half-Bridge Driver/RConn1 -- PWMH/RConn1
  Controlled PWM Voltage/RConn1 -- Half-Bridge Driver/LConn1

== system carpark_shuffler_sim/Power Circuit/Power Shuffler2/Phase B Half Bridge/Phase B Gate Driver ==
  B Control : Inport
  Controlled PWM Voltage : ee_lib/Integrated Circuits/Controlled PWM Voltage  F=200 kHz  TD=1/(2 *200000) s  pulse_width_offset=0 s  pulse_min=0 s  pwm_or_av=ee.enum.pwm_or_av.pwm  event_type=ee.enum.ic.event.asynchronous  sample_time=1e-6 s  Vmin=0 V  Vmax=5 V  Vm=5 V  u_min=0  u_max=1
      settings: InternalSimscapePortConfiguration="{\"Bottom\":[],\"Left\":[{\"id\":\"u\",\"label\":\"u\",\"type\":\"input\"}],\"Right\":[{\"id\":\"p2\",\"label\":\"PWM\",\"type\":\"foundation.electrical.electrical\"},{\"id\":\"n2\",\"label\":\"REF\",\"type\":\"foundation.electrical.electrical\"}],\"Top\":[]}"
  Electrical Reference : fl_lib/Electrical/Electrical Elements/Electrical Reference
  Electrical Reference1 : fl_lib/Electrical/Electrical Elements/Electrical Reference
  Half-Bridge Driver : ee_lib/Semiconductors & Converters/Half-Bridge Driver  port_option=ee.enum.controlport.elec  uHigh=2.0 V  uLow=0.8 V  uHighValue=0.7  uLowValue=0.3  vHigh=15 V  vLow=0 V  tpLH=50 ns  tdLH=100 ns  tpHL=50 ns  tdHL=100 ns  parameterization=ee.enum.semiconductors.gateDriverParam.outputImpedance  rHigh=2 Ohm  rLow=2 Ohm  tRise=20 ns  tFall=20 ns  cLoad=10 nF  ZonTime_specify=off  ZonTime_priority=None  ZonTime=0 s  ZoffTime_specify=off  ZoffTime_priority=None  ZoffTime=0 s  power_dissipated_high_side_specify=off  power_dissipated_high_side_priority=None  power_dissipated_high_side=0 W  power_dissipated_high_side_nominal_specify=off  power_dissipated_high_side_nominal_value=1  power_dissipated_high_side_nominal_unit=W  power_dissipated_low_side_specify=off  power_dissipated_low_side_priority=None  power_dissipated_low_side=0 W  power_dissipated_low_side_nominal_specify=off  power_dissipated_low_side_nominal_value=1  power_dissipated_low_side_nominal_unit=W
      settings: InternalSimscapePortConfiguration="{\"Bottom\":[],\"Left\":[{\"id\":\"PWM\",\"label\":\"PWM\",\"type\":\"foundation.electrical.electrical\"},{\"id\":\"REF\",\"label\":\"REF\",\"type\":\"foundation.electrical.electrical\"}],\"Right\":[{\"id\":\"HO\",\"label\":\"HO\",\"type\":\"foundation.electrical.electrical\"},{\"id\":\"HS\",\"label\":\"HS\",\"type\":\"foundation.electrical.electrical\"},{\"id\":\"LO\",\"label\":\"LO\",\"type\":\"foundation.electrical.electrical\"},{\"id\":\"LS\",\"label\":\"LS\",\"type\":\"foundation.electrical.electrical\"}],\"Top\":[]}"
  Simulink-PS Converter1 : nesl_utility/Simulink-PS Converter  PhysicalDomain=network_engine_domain  SubClassName=ps_input  LeftPortType=input  RightPortType=output  PseudoPeriodic=off  Frequencies=[]  NoiseDistribution=none  NoiseParameters=[]  Unit=1  AffineConversion=off  FilteringAndDerivatives=provide  SimscapeFilterOrder=1  InputFilterTimeConstant=0.001  UdotUserProvided=0
  PWMH : PMIOPort  Side=Right
  phase : PMIOPort  Port=2  Side=Right
  PWML : PMIOPort  Port=3  Side=Right
  wires:
  B Control/1 -> Simulink-PS Converter1/1
  connections:
  Half-Bridge Driver/RConn2 -- phase/RConn1
  Half-Bridge Driver/RConn1 -- PWMH/RConn1
  Half-Bridge Driver/RConn3 -- PWML/RConn1
  Electrical Reference/LConn1 -- Half-Bridge Driver/RConn4
  Simulink-PS Converter1/RConn1 -- Controlled PWM Voltage/LConn1
  Controlled PWM Voltage/RConn1 -- Half-Bridge Driver/LConn1
  Electrical Reference1/LConn1 -- Controlled PWM Voltage/RConn2 -- Half-Bridge Driver/LConn2

== matlab function carpark_shuffler_sim/Supervisor/Recon ==
  data: IL input; IM output; d input
function IM = shuffler_string_recon(IL, d)
%SHUFFLER_STRING_RECON  Module currents from shuffler currents + duties (KCL).
%   What the hardware can compute (no module/string current sensors): module
%   currents RELATIVE to module N (IM(N) = 0). Shuffler k spans modules k,k+1:
%   top terminal node k, midpoint node k+1, bottom terminal node k+2. Averaged
%   per leg: top rail supplies d*iL, bottom rail (1-d)*iL, ic = iLA+iLB into
%   the midpoint. KCL at node j+1 (j = 1..N-1):
%       I_j = I_{j+1} + ic_j - itop_{j+1} - ibot_{j-1}   (out-of-range terms = 0)
%   Inputs: IL (2NS) {ILA1,ILB1,..} in the CONTROL-STACK convention (ILA positive
%   into the midpoint, ILB positive OUT of it, so ILA+ILB = circulating current
%   and ILA-ILB = shuffled current), d (2NS) duties.
%   Stateless; run at the supervisor rate. Mirrors 6_RTOS/ctrl_core/shuffler_recon.c.
%   Validation: (true IM) - IM must be the SAME number for every module.
%#codegen
ILc = IL(:);  dc = d(:);
NS = numel(ILc)/2;  N = NS + 1;
ia = ILc(1:2:end);  ib = -ILc(2:2:end);   % physical B-phase current into the midpoint
da = dc(1:2:end);   db = dc(2:2:end);
itop = da.*ia + db.*ib;
ic   = ia + ib;
ibot = ic - itop;
IM = zeros(N,1);
for j = N-1:-1:1
    acc = IM(j+1) + ic(j);
    if j < NS,  acc = acc - itop(j+1); end
    if j >= 2,  acc = acc - ibot(j-1); end
    IM(j) = acc;
end
end

== matlab function carpark_shuffler_sim/Sensing/MATLAB Function ==
  data: VM input; VMm output; IL input; Vstr input; ILm output; Vstr_m output; SENSE parameter
function [VMm, ILm, Vstr_m] = sense_model(VM, IL, Vstr, SENSE)
%SENSE_MODEL  What the firmware sees (MATLAB Function block source, Sensing subsystem).
%   Sits between the plant's true signals and the Controller/Supervisor so the
%   gains are designed against the board's measurement chain, not ideal signals.
%   Inputs : VM (3) TRUE module voltages, IL (4) TRUE inductor currents in the
%            control-stack convention, Vstr TRUE string voltage at the load.
%   Param  : SENSE (struct from init_params, scope = Parameter).
%   Outputs: VMm (3) module voltages as formed in App/app.c, ILm (4) as from
%            Core/Src/sensors.c, Vstr_m the e-load readback the Pi would forward.
%   Block sample time: SENSE.Ts (100e-6), atomic.
%
%   Voltages: three INA239 bus readings, refreshed every SENSE.ina_div ticks
%     U12 = VM3            (CS1)
%     U11 = VM2 + VM3      (CS2)
%     U10 = VM1 + VM2      (CS3, PV1+ to PV3+, behind the ISO7762)
%   quantised to 3.125 mV, then VM3 = U12, VM2 = U11 - U12 and VM1 from SENSE.vm1_src:
%     0 INA         VM1 = U10 - VM2
%     1 VSTR_PARAM  VM1 = vstr_param - VM2 - VM3   (e-load CV setpoint, full rate)
%     2 VSTR_PI     VM1 = Vstr_m - VM2 - VM3       (e-load readback, ~2.2 Hz, held)
%   Currents: averaged plant -> the tick-mean is the sample; quantised on the 12-bit
%   ADC through the FITTED sensitivity and converted back with the FIRMWARE's one,
%   so kX_hw ~= kX_fw reproduces a scaling error.
%#codegen
persistent n_ina n_pi U Vpi
if isempty(n_ina)
    n_ina = 0;  n_pi = 0;  U = zeros(3,1);  Vpi = Vstr;
end
VMc = VM(:);  ILc = IL(:);

% ---- INA239 round robin (1 kHz) ----
if n_ina == 0
    Ut = [VMc(3); VMc(2) + VMc(3); VMc(1) + VMc(2)];
    if SENSE.noise_vm > 0, Ut = Ut + SENSE.noise_vm * randn(3,1); end
    U = SENSE.ina_lsb * round(Ut / SENSE.ina_lsb);
end
n_ina = n_ina + 1;
if n_ina >= SENSE.ina_div, n_ina = 0; end

% ---- e-load readback through the Pi ----
if n_pi == 0
    Vpi = SENSE.vstr_lsb * round(Vstr / SENSE.vstr_lsb);
end
n_pi = n_pi + 1;
if n_pi >= SENSE.vstr_pi_div, n_pi = 0; end
Vstr_m = Vpi;

VMm = zeros(3,1);
VMm(3) = U(1);
VMm(2) = U(2) - U(1);
switch SENSE.vm1_src
    case 1
        VMm(1) = SENSE.vstr_param - VMm(2) - VMm(3);
    case 2
        VMm(1) = Vpi - VMm(2) - VMm(3);
    otherwise
        VMm(1) = U(3) - VMm(2);
end

% ---- hall + ADC ----
khw = [SENSE.kA_hw; SENSE.kB_hw; SENSE.kA_hw; SENSE.kB_hw];
kfw = [SENSE.kA_fw; SENSE.kB_fw; SENSE.kA_fw; SENSE.kB_fw];
It = ILc;
if SENSE.noise_il > 0, It = It + SENSE.noise_il * randn(4,1); end
counts = min(max(round(It .* khw / SENSE.adc_lsb), -2048), 2047);   % 1.65 V mid-rail, 12-bit
ILm = counts * SENSE.adc_lsb ./ kfw;
end

== matlab function carpark_shuffler_sim/Controller/Controller ==
  data: VM input; d output; IL input; rv input; CTRL parameter
function d = shuffler_string_ctrl(VM, IL, rv, CTRL)
%SHUFFLER_STRING_CTRL  Inner decoupling-PI controller (MATLAB Function block source).
%   Generic in the module count: N = numel(VM), NS = N-1 shufflers.
%   Inputs : VM (N x 1) module voltages AS MEASURED, IL (2NS x 1) {ILA1,ILB1,ILA2,ILB2,..}
%            in the control-stack convention (ILA into the midpoint, ILB out of it),
%            rv (NS x 1) voltage-difference references.
%   Param  : CTRL (struct from init_params, scope = Parameter in the block's
%            Ports and Data Manager - no port): Ts, M, Kp_ratio, fc, DMIN, DMAX, kscale.
%   Output : d (2NS x 1) duties {dA1,dB1,dA2,dB2,..} clamped to [DMIN,DMAX].
%   Block sample time: CTRL.Ts (explicit, atomic). Mirrors 6_RTOS/ctrl_core/shuffler_ctrl.c;
%   kscale mirrors the firmware runtime gain scale (Mp and M scaled, Minv by 1/kscale).
%#codegen
N  = numel(VM);  NS = N - 1;
Ts = CTRL.Ts;
M    = CTRL.kscale * CTRL.M;
Mp   = M * diag(CTRL.Kp_ratio);
Minv = inv(M);                      % recomputed each call: tunable CTRL survives Fast Restart
a    = 2*pi*CTRL.fc*Ts / (1 + 2*pi*CTRL.fc*Ts);
persistent xi y_f
if isempty(xi)
    xi = zeros(2*NS,1); y_f = zeros(2*NS,1);
end
VMc = VM(:);  ILc = IL(:);
y   = [VMc(1:NS) - VMc(2:N); ILc(1:2:end) + ILc(2:2:end)];
y_f = y_f + a*(y - y_f);
r   = [rv(:); zeros(NS,1)];
e   = r - y_f;
xi_try = xi + Ts*e;
u      = Mp*e + M*xi_try;
uc = u(1:NS);  ud = u(NS+1:2*NS);
dA = 0.5 + 0.5*(uc + ud);
dB = 0.5 + 0.5*(uc - ud);
dAs = min(max(dA, CTRL.DMIN), CTRL.DMAX);
dBs = min(max(dB, CTRL.DMIN), CTRL.DMAX);
u_act = [(dAs + dBs) - 1; dAs - dBs];
xi    = Minv * (u_act - Mp*e);
d = zeros(2*NS,1);
d(1:2:end) = dAs;
d(2:2:end) = dBs;
end

== matlab function carpark_shuffler_sim/Supervisor/Supervisor ==
  data: VM input; rv output; IM input; IL input; d input; en input; beta output; stress output
function [rv, beta, stress] = shuffler_string_supervisor(VM, IM, IL, d, en)
%SHUFFLER_STRING_SUPERVISOR  Feasibility governor (MATLAB Function block source).
%   Generic in N = numel(IM). IM may be ABSOLUTE (plant) or RELATIVE (recon
%   block): only max(imf) - imf is used, so a common offset cancels.
%   Inputs : VM (N) unused, IM (N), IL (2NS), d (2NS) applied duties, en.
%   Outputs: rv (NS x 1) relaxation refs, beta, stress. Sample time 1e-3, atomic.
%   Mirrors 6_RTOS/ctrl_core/shuffler_supervisor.c.
%#codegen
N = numel(IM);  NS = N - 1;  %#ok<NASGU>
ILc = IL(:);  IMc = IM(:);  dc = d(:);
id = ILc(1:2:end) - ILc(2:2:end);
Ts3 = 1e-3;  TF = 5e-3;  I_RATED = 10;
S_HI = 0.90;  S_LO = 0.70;  KB = 60;  KREL = 6;  BMAX = 4;  RVMAX = 30;
persistent b imf idf
if isempty(b), b = 0; imf = IMc; idf = id; end
if en == 0
    b = 0; imf = IMc; idf = id;
    rv = zeros(N-1,1); beta = 0; stress = 0; return;
end
imf = imf + (Ts3/TF)*(IMc - imf);
dl  = max(imf) - imf;
idf = idf + (Ts3/TF)*(id - idf);
stress = max( max(abs(idf))/I_RATED , max(abs(dc - 0.5))/0.45 );
if stress > S_HI
    b = b + Ts3*KB*(stress - S_HI);
elseif stress < S_LO
    b = b - Ts3*KREL*(S_LO - stress);
end
b = min(max(b,0), BMAX);
rv = b*(dl(2:N) - dl(1:N-1));
rv = min(max(rv,-RVMAX), RVMAX);
beta = b;
end

== matlab function carpark_shuffler_sim/MPPT/P&O ==
  data: Vstr input; Iref output; Istr input; beta input; en input; Pav output; state output
function [Iref, Pav, state] = shuffler_string_mppt(Vstr, Istr, beta, en)
%#codegen
% SHUFFLER_STRING_MPPT  Adaptive-step P&O on the STRING CURRENT.
%   Sits above the governor: perturbs the load current sink's reference I_ref,
%   measures string power averaged over each perturb window, and climbs.
%   The DPP-equalised string has a UNIMODAL P-V curve (the shufflers remove the
%   multi-peak problem), so a hill climber is sufficient by construction.
%
%   Adaptive step: |step| = clip(KA*|dP|, SMIN, SMAX) -> big steps far from the
%   peak, small steps near it. Deadband DB parks it at the top (no dither).
%   Governor hold-off: while the supervisor's beta is MOVING, P is being changed
%   by protection, not by us -> freeze and re-baseline (never climb on a
%   confounded measurement). A parked (constant) beta, even nonzero, is fine.
%
%   Block sample time Ts = 1e-3. One perturb decision every TP seconds.
%
%   Inputs : Vstr  string voltage (N0-N4, or sum VM1..4)             [V]
%            Istr  string current (sensor at the sink)               [A]
%            beta  supervisor governor state (hold-off signal)      [V/A]
%            en    enable (0 -> hold IREF0, reset)
%   Outputs: Iref  command for the controlled-current-sink load      [A]
%            Pav   last windowed power measurement (scope it)        [W]
%            state 0 = holding (governor active/boot), 1 = climbing, 2 = parked

Ts    = 1e-3;      % this block's sample time [s]
TP    = 0.02;      % perturb period [s] (string settles in ~ms; 50 ms is generous)
IREF0 = 12;        % initial string current [A] (below MPP ~14.35 -> climbs up)
IMIN  = 5;         % lower clamp [A]
IMAX  = 14.5;      % upper clamp [A] — keep BELOW the strong modules' Isc (14.96):
                   %   above Isc the string voltage collapses; don't let P&O visit
DB    = 1.0;       % power deadband [W]: |dP| below this -> parked, no step
KA    = 0.01;      % adaptive step gain [A/W]
SMIN  = 0.05;      % step clamp [A]
SMAX  = 1.0;
S0    = 0.25;      % bootstrap first-step size [A]
BTOL  = 1e-3;      % beta movement per window that counts as "governor active"

N = round(TP/Ts); % samples per perturb window

persistent iref dirn Pprev acc n boot b0 st
if isempty(iref)
    iref=IREF0; dirn=1; Pprev=0; acc=0; n=0; boot=true; b0=beta; st=0;
end

if en == 0
    iref=IREF0; dirn=1; Pprev=0; acc=0; n=0; boot=true; b0=beta; st=0;
    Iref=iref; Pav=Vstr*Istr; state=0; return;
end

% ---- accumulate power over the perturb window ----
acc = acc + Vstr*Istr;
n   = n + 1;

if n >= N
    Pw  = acc/N;  acc = 0;  n = 0;
    govActive = abs(beta - b0) > BTOL;   b0 = beta;

    if govActive
        boot = true;  st = 0;            % protection is moving the plant:
                                          % freeze, re-baseline when it parks
    elseif boot
        Pprev = Pw;  boot = false;       % baseline window, then a first nudge
        iref  = iref + dirn*S0;  st = 1;
    else
        dP = Pw - Pprev;
        if dP > DB                        % better -> keep going, scaled step
            step = min(max(KA*abs(dP),SMIN),SMAX);
            iref = iref + dirn*step;  st = 1;
        elseif dP < -DB                   % worse -> reverse, scaled step
            dirn = -dirn;
            step = min(max(KA*abs(dP),SMIN),SMAX);
            iref = iref + dirn*step;  st = 1;
        else                              % inside deadband -> parked at MPP
            st = 2;
        end
        Pprev = Pw;                       % always track (follows irradiance)
    end
    iref = min(max(iref,IMIN),IMAX);
end

Iref  = iref;
Pav   = Pprev;
state = st;
end
